simulink model "dc1_op_unlinked_R2016a"  (R2016a)
settings: Solver=FixedStepDiscrete  StartTime=0.0  StopTime=2.5  RelTol=1e-3
InitFcn:
  | Ts_Control=100e-6;
  | Ts_Power=Ts_Control/50;
undefined symbols (not defined in the file): TeN
libraries: powerlib x12, powerlib_meascontrol x3
Description:
  | Copyright 2008-2017 The MathWorks, Inc.
settings Model: ExtModeAutoUpdateStatusClock=off  Creator=MathWorks  LastModifiedBy=CX
settings DataIOCC: LimitDataPoints=on  SaveFormat=Array  SignalLoggingSaveFormat=ModelDataLogs  SaveOutput=off  SignalLogging=off  SaveTime=off  SignalLoggingName=sigsOut
settings OptimizationCC: ExpressionDepthLimit=2147483647  InitFltsAndDblsToZero=on
settings DebuggingCC: UnderspecifiedInitializationDetection=Classic  MergeDetectMultiDrivingBlocksExec=none  CheckExecutionContextPreStartOutputMsg=on  CheckExecutionContextRuntimeOutputMsg=on  SignalResolutionControl=TryResolveAllWithWarning  MultiTaskDSMMsg=warning  MultiTaskCondExecSysMsg=none  FcnCallInpInsideContextMsg=EnableAllAsWarning  StateNameClashWarn=warning
settings HardwareCC: ProdBitPerPointer=32  ProdLargestAtomicFloat=None  ProdIntDivRoundTo=Undefined  ProdEndianess=Unspecified  ProdWordSize=32  ProdHWDeviceType=32-bit Generic  TargetUnknown=on
settings ModelReferenceCC: PropagateSignalLabelsOutOfModel=off
settings GRTTargetCC: CombineOutputUpdateFcns=off  GRTInterface=on
settings ConfigComp: CovSFcnEnable=off
settings SimscapeCC: SimscapeNormalizeSystem=off

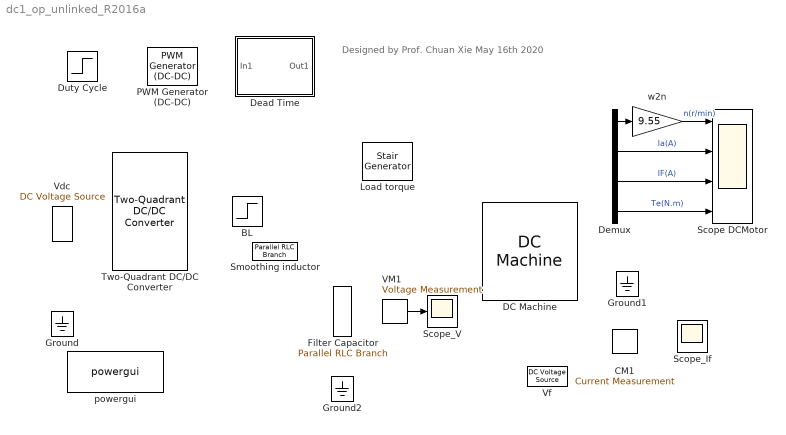
== system dc1_op_unlinked_R2016a ==
  note: Designed by Prof. Chuan Xie
      | May 16th 2020
  BL : Step  Time=0.2  Before=1  After=0  SampleTime=Ts_Power
  CM1 : powerlib/Measurements/Current Measurement  PhasorSimulation=off  OutputType=Complex  PSBequivalent=0
  DC Machine : powerlib/Machines/DC Machine  PresetModel=02: 5HP 240V 1750RPM Field:150V  MechanicalLoad=Torque TL  FieldType=Wound  ShowDetailedParameters=on  MeasurementBus=off  RLa=[0.78 0.016]  RLf=[150 112.5]  Laf=1.234  MachineConstant=Torque constant (N.m/A)  Ke=1.8  Kt=1.8  J=0.05  Bm=0.01  Tf=0  w0=1800/9.55  Ifinit=1  TsPowergui=0  TsBlock=-1
  Dead Time : Subsystem
  Demux : Demux
  Duty Cycle : Step  Time=0.1  After=0.8  SampleTime=Ts_Power
  Filter Capacitor : powerlib/Elements/Parallel RLC Branch  LConnTagsString=a  RConnTagsString=__new0  BranchType=C  Resistance=[]  Inductance=0.5e-3  SetiL0=off  InitialCurrent=0  Capacitance=100e-6  Setx0=off  InitialVoltage=0  Measurements=None
  Ground : powerlib/Elements/Ground  LConnTagsString=a
  Ground1 : powerlib/Elements/Ground  LConnTagsString=a
  Ground2 : powerlib/Elements/Ground  LConnTagsString=a
  Load torque : powerlib_meascontrol/Pulse & Signal Generators/Stair Generator  t=[0, 0.5, 1, 1.5 2]  e=[1, 0.75, 0.5, 0.25, 0.1]*TeN  Ts=0
  PWM Generator (DC-DC) : powerlib_meascontrol/Pulse & Signal Generators/PWM Generator (DC-DC)  Fsw=10e3  Ts=Ts_Power
  Scope DCMotor : Scope  NumInputPorts=4
  Scope_If : Scope
  Scope_V : Scope
  Smoothing inductor : powerlib/Elements/Parallel RLC Branch  LConnTagsString=a  RConnTagsString=__new0  BranchType=L  Resistance=[]  Inductance=5e-3  SetiL0=off  InitialCurrent=0  Capacitance=[]  Setx0=off  InitialVoltage=0  Measurements=None
  Two-Quadrant DC/DC Converter : powerlib/Power Electronics/Two-Quadrant DC//DC Converter  ModelType=Switching devices  Ron=0.5  Rs=1e6  Cs=inf  Vforward=[0,0]  Ron_Diode=1e-3  Rs_Diode=1e6  Cs_Diode=inf  Vf_Diode=1e-3  Rs_CurrentSource=inf
  VM1 : powerlib/Measurements/Voltage Measurement  PhasorSimulation=off  OutputType=Complex  PSBequivalent=0
  Vdc : powerlib/Electrical Sources/DC Voltage Source  Description=source block  Amplitude=300  Measurements=None
      settings: AttributesFormatString=\n
  Vf : powerlib/Electrical Sources/DC Voltage Source  Description=source block  Amplitude=150  Measurements=None
      settings: AttributesFormatString=\n
  powergui : powerlib/powergui  Priority=2  SimulationMode=Discrete  SampleTime=Ts_Power  frequency=60  Iterations=50  frequencyindice=0  Pbase=100e6  ErrMax=1e-4  UnitsV=kV  UnitsW=MW  buscounter=0  FunctionMessages=off  echomessages=off  EnableUseOfTLC=off  CurrentSourceSwitches=off  DisableSnubberDevices=off  DisableRonSwitches=off  DisableVfSwitches=off  DisplayEquations=off  SolverType=Tustin/Backward Euler (TBE)  Interpol=off  ExternalGateDelay=off  methode=off  Ts=0  x0status=blocks  SPID=off  SwTol=0  HookPort=off  RestoreLinks=warning  ResistiveCurrentMeasurement=off  Frange=[0:2:500]  Ylog=off  Xlog=on  ShowGrid=off  save=off  variable=ZData  structure=0  ZoomFFT=on  StartTime=0.0  cycles=1  DisplayStyle=1  fundamental=60  FreqAxis=off  MaxFrequency=1000  frequencyindicesteady=1  RmsSteady=1  display=off
  w2n : Gain  Gain=9.55
  wires:
  Demux/1 -> w2n/1
  Demux/2 -> Scope DCMotor/2  "Ia(A)"
  Demux/3 -> Scope DCMotor/3  "IF(A)"
  Demux/4 -> Scope DCMotor/4  "Te(N.m)"
  w2n/1 -> Scope DCMotor/1  "n(r/min)"
  VM1/1 -> Scope_V/1

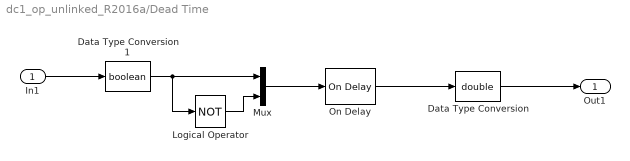
== system dc1_op_unlinked_R2016a/Dead Time ==
  In1 : Inport
  Data Type Conversion : DataTypeConversion  OutDataTypeStr=double
  Data Type Conversion1 : DataTypeConversion  OutDataTypeStr=boolean
  Logical Operator : Logic  Operator=NOT  AllPortsSameDT=off  OutDataTypeStr=boolean
  Mux : Mux  Inputs=2
  On Delay : powerlib_meascontrol/Logic/On Delay  DelayType=On delay  delay=Ts_Power*2  ic=0  Ts=Ts_Power
  Out1 : Outport
  wires:
  In1/1 -> Data Type Conversion1/1
  Logical Operator/1 -> Mux/2
  On Delay/1 -> Data Type Conversion/1
  Mux/1 -> On Delay/1
  Data Type Conversion1/1 -> Logical Operator/1, Mux/1
  Data Type Conversion/1 -> Out1/1
